simulink model "tb_per_scanfilter"  (R2026b)
undefined symbols (not defined in the file or in its folder): Ts
settings Model: Creator=aomar  LastModifiedBy=aomar

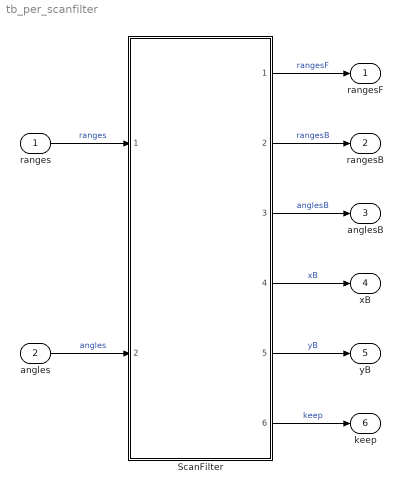
== system tb_per_scanfilter ==
  ranges : Inport  OutDataTypeStr=single  PortDimensions=P.sensors.lidar.nBeams  SampleTime=Ts.perception  Interpolate=off
  angles : Inport  Port=2  OutDataTypeStr=single  PortDimensions=P.sensors.lidar.nBeams  SampleTime=Ts.perception  Interpolate=off
  ScanFilter : Subsystem  ReferencedSubsystem=sens_scan_filter
  rangesF : Outport
  rangesB : Outport  Port=2
  anglesB : Outport  Port=3
  xB : Outport  Port=4
  yB : Outport  Port=5
  keep : Outport  Port=6
  wires:
  ranges/1 -> ScanFilter/1  "ranges"
  angles/1 -> ScanFilter/2  "angles"
  ScanFilter/1 -> rangesF/1  "rangesF"
  ScanFilter/2 -> rangesB/1  "rangesB"
  ScanFilter/3 -> anglesB/1  "anglesB"
  ScanFilter/4 -> xB/1  "xB"
  ScanFilter/5 -> yB/1  "yB"
  ScanFilter/6 -> keep/1  "keep"
